simulink model "motion_controller"  (R2025b)
settings: configuration reference "MCConfiguration" (kept outside this file)
undefined symbols (not defined in the file): EstimationVelocityModes, Ts_ControlOuter, Ts_MotionController
settings Model: DataDictionary=embeddedBoard_common.sldd  VariantConfigurationObject=MCVariants  SimulationMode=accelerator  Creator=mfussi  LastModifiedBy=rpumpo
settings ConfigSetRef: SourceName=MCConfiguration

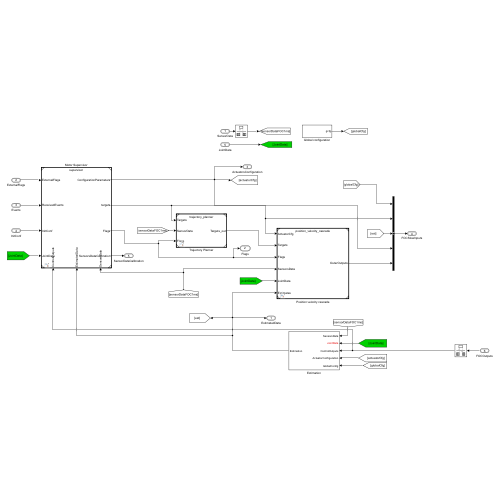
[thumbnail: Simulink's stored preview of the top-level diagram]
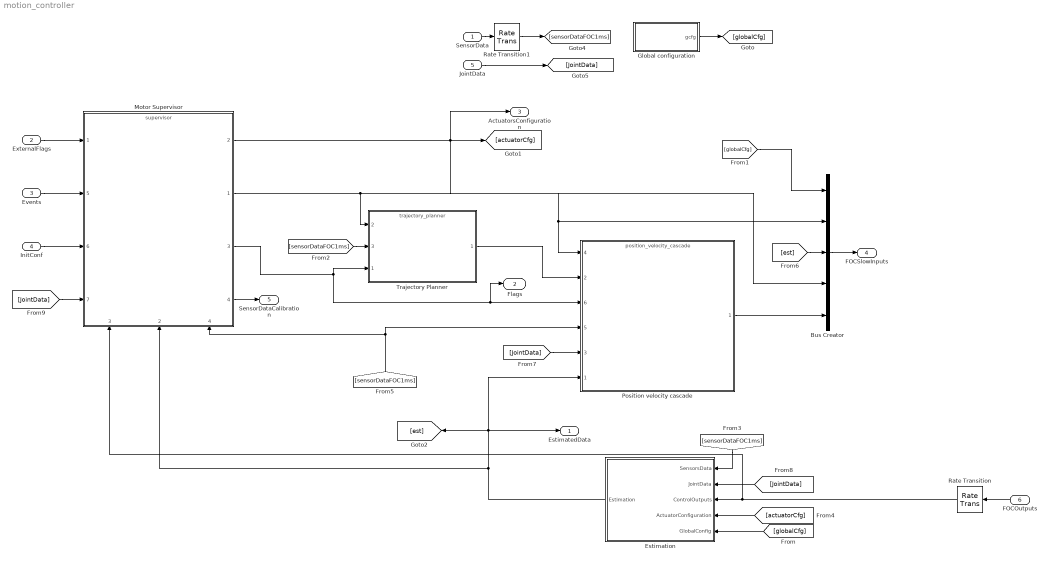
== system motion_controller ==
  SensorData : Inport  OutDataTypeStr=Bus: SensorsData  BusOutputAsStruct=on
  ExternalFlags : Inport  Port=2  OutDataTypeStr=Bus: ExternalFlags  BusOutputAsStruct=on
  Events : Inport  Port=3  OutDataTypeStr=Bus: ReceivedEvents  PortDimensions=MAX_EVENTS_PER_TICK  BusOutputAsStruct=on
  InitConf : Inport  Port=4  OutDataTypeStr=Bus: ActuatorConfiguration  BusOutputAsStruct=on
  JointData : Inport  Port=5  OutDataTypeStr=Bus: JointData  SampleTime=Ts_ControlOuter  BusOutputAsStruct=on
  FOCOutputs : Inport  Port=6  OutDataTypeStr=Bus: FOCOutputs  BusOutputAsStruct=on
  Bus Creator : BusCreator  Inputs=5  OutDataTypeStr=Bus: FOCSlowInputs  NonVirtualBus=on
      settings: InheritFromInputs=off
  Estimation : Subsystem
  Global configuration : Subsystem
  Motor Supervisor : ModelReference  ModelNameDialog=supervisor.slx  SimulationMode=Normal  ModelReferenceVersion=5.31
      settings: PortSchema="{\"entries\":[{\"content\":{\"sides\":[{\"content\":{\"connectorIds\":[\"In1\",\"In5\",\"In6\",\"In7\"]},\"type\":\"ConnectorPlacement.EquallySpacedRectSide\",\"uuid\":\"cef8e8ad-9c58-41ab-a08a-9ae722e40085\"},{\"content\":{\"connectorIds\":[\"Out2\",\"Out1\",\"Out3\",\"Out4\"],\"side\":\"RIGHT\"},\"type\":\"ConnectorPlacement.EquallySpacedRectSide\",\"uuid\":\"f0f6bf4d-d146-4c52-85d0-e4a1fe2e14c9\"},{\"content\":{\"side\":\"TOP\"},\"type\":\"ConnectorPlacement.EquallySpacedRectSide\",\"uuid\":\"118dcde8-f32d-4dec-aaf2-5a7aa823a04d\"},{\"content\":{\"connectorIds\":[\"In3\",\"In2\",\"In4\"],\"side\":\"BOTTOM\"},\"type\":\"ConnectorPlacement.EquallySpacedRectSide\",\"uuid\":\"c7cf3ffe-4331-4ad3-8d42-678750b74e71\"}]},\"type\":\"ConnectorPlacement.EquallySpacedConnector\",\"uuid\":\"5370414b-b8cf-4747-9f7c-0256206e2ab5\"}],\"packageUris\":[\"http://schema.mathworks.com/mf0/Connector/R2020b\"],\"version\":\"1.0\"}"
  Position velocity cascade : ModelReference  ModelNameDialog=position_velocity_cascade.slx  SimulationMode=Normal  ModelReferenceVersion=10.15
      settings: PortSchema="{\"entries\":[{\"content\":{\"sides\":[{\"content\":{\"connectorIds\":[\"In4\",\"In2\",\"In6\",\"In5\",\"In3\",\"In1\"]},\"type\":\"ConnectorPlacement.EquallySpacedRectSide\",\"uuid\":\"5f0855f7-78ef-4761-b7b2-78e76d92fc4b\"},{\"content\":{\"connectorIds\":[\"Out1\"],\"side\":\"RIGHT\"},\"type\":\"ConnectorPlacement.EquallySpacedRectSide\",\"uuid\":\"ce4374cd-607c-4e0b-a8af-eb2e0e17051d\"},{\"content\":{\"side\":\"TOP\"},\"type\":\"ConnectorPlacement.EquallySpacedRectSide\",\"uuid\":\"cef85d5e-e838-4f2a-8e72-80e83911c8d3\"},{\"content\":{\"side\":\"BOTTOM\"},\"type\":\"ConnectorPlacement.EquallySpacedRectSide\",\"uuid\":\"20390ec2-cce8-49cd-a78c-2a21c95dd133\"}]},\"type\":\"ConnectorPlacement.EquallySpacedConnector\",\"uuid\":\"234d6756-2ddf-48d1-9c55-249229e32550\"}],\"packageUris\":[\"http://schema.mathworks.com/mf0/Connector/R2020b\"],\"version\":\"1.0\"}"
  Rate Transition : RateTransition  Deterministic=off  OutPortSampleTime=Ts_Supervision
  Rate Transition1 : RateTransition  Deterministic=off  OutPortSampleTime=Ts_Supervision
  Trajectory Planner : ModelReference  ModelNameDialog=trajectory_planner.slx  SimulationMode=Normal  ModelReferenceVersion=2.33
      settings: PortSchema="{\"entries\":[{\"content\":{\"sides\":[{\"content\":{\"connectorIds\":[\"In2\",\"In3\",\"In1\"]},\"type\":\"ConnectorPlacement.EquallySpacedRectSide\",\"uuid\":\"9df5b159-43e0-4cee-9566-6165d3b4308e\"},{\"content\":{\"connectorIds\":[\"Out1\"],\"side\":\"RIGHT\"},\"type\":\"ConnectorPlacement.EquallySpacedRectSide\",\"uuid\":\"a479e708-d845-4af6-a357-888a4bbec164\"},{\"content\":{\"side\":\"TOP\"},\"type\":\"ConnectorPlacement.EquallySpacedRectSide\",\"uuid\":\"08bafdfa-e50b-4564-8577-557c5ee22102\"}]},\"type\":\"ConnectorPlacement.EquallySpacedConnector\",\"uuid\":\"f51dce5d-e2ef-40ca-b0ed-04a94a0f54f0\"}],\"packageUris\":[\"http://schema.mathworks.com/mf0/Connector/R2020b\"],\"version\":\"1.0\"}"
  EstimatedData : Outport  OutDataTypeStr=Bus: EstimatedData  BusOutputAsStruct=on
  Flags : Outport  Port=2  OutDataTypeStr=Bus: Flags  BusOutputAsStruct=on
  ActuatorsConfiguration : Outport  Port=3  OutDataTypeStr=Bus: ActuatorConfiguration  BusOutputAsStruct=on
  FOCSlowInputs : Outport  Port=4  OutDataTypeStr=Bus: FOCSlowInputs  BusOutputAsStruct=on
  SensorDataCalibration : Outport  Port=5  OutDataTypeStr=Bus: SensorsData  BusOutputAsStruct=on
  wires:
  Bus Creator/1 -> FOCSlowInputs/1
  Events/1 -> Motor Supervisor/5
  Motor Supervisor/1 -> Trajectory Planner/2, Bus Creator/4
  [actuatorCfg] -> Estimation/4(ActuatorConfiguration)
  FOCOutputs/1 -> Rate Transition/1
  Global configuration/1(gcfg) -> [globalCfg]
  Position velocity cascade/1 -> Bus Creator/5
  [globalCfg] -> Estimation/5(GlobalConfig)
  [globalCfg] -> Bus Creator/1
  InitConf/1 -> Motor Supervisor/6
  Motor Supervisor/2 -> ActuatorsConfiguration/1, [actuatorCfg], Position velocity cascade/4, Bus Creator/2
  ExternalFlags/1 -> Motor Supervisor/1
  [est] -> Bus Creator/3
  Motor Supervisor/3 -> Flags/1, Position velocity cascade/6, Trajectory Planner/1
  Estimation/1(Estimation) -> EstimatedData/1, Position velocity cascade/1, [est], Motor Supervisor/2
  SensorData/1 -> Rate Transition1/1
  [sensorDataFOC1ms] -> Position velocity cascade/5, Motor Supervisor/4
  [sensorDataFOC1ms] -> Estimation/1(SensorsData)
  JointData/1 -> [JointData]
  [JointData] -> Position velocity cascade/3
  [JointData] -> Estimation/2(JointData)
  [JointData] -> Motor Supervisor/7
  Rate Transition1/1 -> [sensorDataFOC1ms]
  Rate Transition/1 -> Motor Supervisor/3, Estimation/3(ControlOutputs)
  Motor Supervisor/4 -> SensorDataCalibration/1
  [sensorDataFOC1ms] -> Trajectory Planner/3
  Trajectory Planner/1 -> Position velocity cascade/2

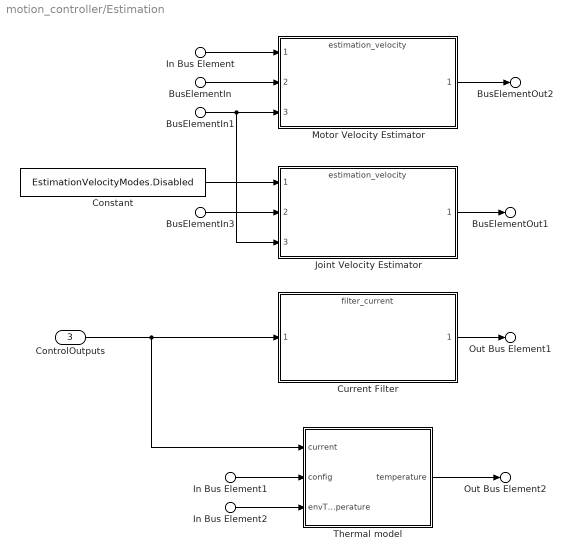
== system motion_controller/Estimation ==
  BusElementIn : Inport  Description=Mechanical Angle before gearbox  PortName=SensorsData  Element=motorsensors.qencoder.rotor_angle
  BusElementIn3 : Inport  Description=position encoder after gearbox  Port=2  PortName=JointData  Element=position
  ControlOutputs : Inport  Port=3  OutDataTypeStr=Bus: FOCOutputs
  In Bus Element1 : Inport  Port=4  PortName=ActuatorConfiguration  Element=motor
  In Bus Element2 : Inport  Port=5  PortName=GlobalConfig  Element=estimation.environment_temperature
  In Bus Element : Inport  Port=5  PortName=GlobalConfig  Element=estimation.velocity_est_mode
  BusElementIn1 : Inport  Port=5  PortName=GlobalConfig  Element=estimation.velocity_est_window
  Constant : Constant  Value=EstimationVelocityModes.Disabled  OutDataTypeStr=Enum: EstimationVelocityModes
  Current Filter : ModelReference  ModelNameDialog=filter_current.slx  SimulationMode=Normal  ModelReferenceVersion=8.0
  Joint Velocity Estimator : ModelReference  ModelNameDialog=estimation_velocity.slx  SimulationMode=Normal  ModelReferenceVersion=8.11
  Motor Velocity Estimator : ModelReference  ModelNameDialog=estimation_velocity.slx  SimulationMode=Normal  ModelReferenceVersion=8.11
  Thermal model : Subsystem  Variant=on
  BusElementOut2 : Outport  Description=velocity  PortName=Estimation  Element=rotor_velocity
  Out Bus Element1 : Outport  Description=filtered motor current  PortName=Estimation  Element=Iq_filtered
  Out Bus Element2 : Outport  Description=motor temperature  PortName=Estimation  Element=motor_temperature
  BusElementOut1 : Outport  Description=velocity  PortName=Estimation  Element=joint_velocity
  wires:
  Motor Velocity Estimator/1 -> BusElementOut2/1
  Current Filter/1 -> Out Bus Element1/1
  ControlOutputs/1 -> Current Filter/1, Thermal model/1(current)
  In Bus Element/1 -> Motor Velocity Estimator/1
  In Bus Element1/1 -> Thermal model/2(config)
  In Bus Element2/1 -> Thermal model/3(envTemperature)
  Thermal model/1(temperature) -> Out Bus Element2/1
  BusElementIn/1 -> Motor Velocity Estimator/2
  BusElementIn1/1 -> Joint Velocity Estimator/3, Motor Velocity Estimator/3
  BusElementIn3/1 -> Joint Velocity Estimator/2
  Joint Velocity Estimator/1 -> BusElementOut1/1
  Constant/1 -> Joint Velocity Estimator/1

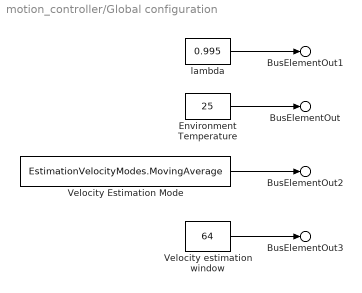
== system motion_controller/Global configuration ==
  Environment Temperature : Constant  Value=25  OutDataTypeStr=single  SampleTime=Ts_MotionController
  Velocity Estimation Mode : Constant  Value=EstimationVelocityModes.MovingAverage  OutDataTypeStr=Enum: EstimationVelocityModes  SampleTime=Ts_MotionController
  Velocity estimation window : Constant  Value=64  OutMin=1  OutDataTypeStr=uint32  SampleTime=Ts_MotionController
  lambda : Constant  Value=0.995  OutDataTypeStr=single  SampleTime=Ts_MotionController
  BusElementOut : Outport  PortName=gcfg  Element=estimation.environment_temperature
  BusElementOut1 : Outport  PortName=gcfg  Element=estimation.current_rms_lambda
  BusElementOut2 : Outport  PortName=gcfg  Element=estimation.velocity_est_mode
  BusElementOut3 : Outport  PortName=gcfg  Element=estimation.velocity_est_window
  wires:
  lambda/1 -> BusElementOut1/1
  Velocity Estimation Mode/1 -> BusElementOut2/1
  Velocity estimation window/1 -> BusElementOut3/1
  Environment Temperature/1 -> BusElementOut/1

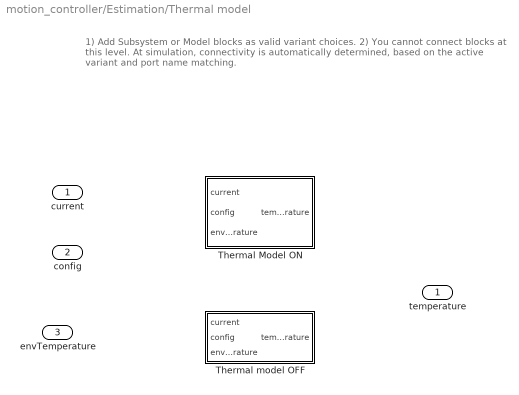
== system motion_controller/Estimation/Thermal model ==
  note: 1) Add Subsystem or Model blocks as valid variant choices.
      | 2) You cannot connect blocks at this level. At simulation, connectivity is automatically
      | determined, based on the active variant and port name matching.
  current : Inport
  config : Inport  Port=2
  envTemperature : Inport  Port=3
  Thermal Model ON : Subsystem  VariantControl=Temperature_estimation_switch == true
  Thermal model OFF : Subsystem  VariantControl=Temperature_estimation_switch == false
  temperature : Outport

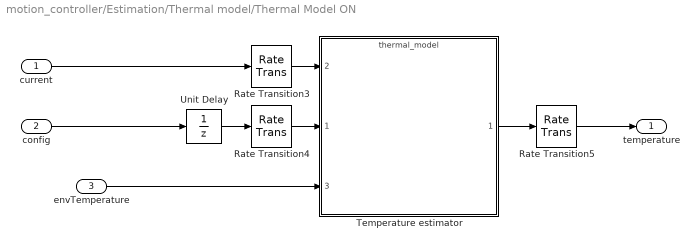
== system motion_controller/Estimation/Thermal model/Thermal Model ON ==
  current : Inport
  config : Inport  Port=2
  envTemperature : Inport  Port=3
  Rate Transition3 : RateTransition  Deterministic=off
  Rate Transition4 : RateTransition  Deterministic=off  OutPortSampleTime=1e-3
  Rate Transition5 : RateTransition  Deterministic=off
  Temperature estimator : ModelReference  ModelNameDialog=thermal_model.slx  SimulationMode=Normal  ModelReferenceVersion=8.0
      settings: PortSchema="{\"entries\":[{\"content\":{\"sides\":[{\"content\":{\"connectorIds\":[\"In2\",\"In1\",\"In3\"]},\"type\":\"ConnectorPlacement.EquallySpacedRectSide\",\"uuid\":\"78c786f4-5c3b-40e7-ad28-c0b961f14ec4\"},{\"content\":{\"connectorIds\":[\"Out1\"],\"side\":\"RIGHT\"},\"type\":\"ConnectorPlacement.EquallySpacedRectSide\",\"uuid\":\"b3487c62-68f2-43b6-a257-d51b1fb2e448\"},{\"content\":{\"side\":\"TOP\"},\"type\":\"ConnectorPlacement.EquallySpacedRectSide\",\"uuid\":\"5ce4df9e-b156-438c-989b-62dab6cef7f1\"}]},\"type\":\"ConnectorPlacement.EquallySpacedConnector\",\"uuid\":\"8f8c8caf-b0d2-4a2e-a596-6a6abf765763\"}],\"packageUris\":[\"http://schema.mathworks.com/mf0/Connector/R2020b\"],\"version\":\"1.0\"}"
  Unit Delay : UnitDelay  SampleTime=-1  HasFrameUpgradeWarning=on
  temperature : Outport
  wires:
  Rate Transition4/1 -> Temperature estimator/1
  config/1 -> Unit Delay/1
  Unit Delay/1 -> Rate Transition4/1
  Temperature estimator/1 -> Rate Transition5/1
  current/1 -> Rate Transition3/1
  Rate Transition3/1 -> Temperature estimator/2
  Rate Transition5/1 -> temperature/1
  envTemperature/1 -> Temperature estimator/3

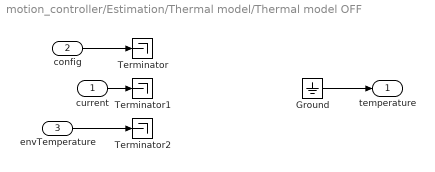
== system motion_controller/Estimation/Thermal model/Thermal model OFF ==
  current : Inport
  config : Inport  Port=2
  envTemperature : Inport  Port=3
  Ground : Ground
  Terminator : Terminator
  Terminator1 : Terminator
  Terminator2 : Terminator
  temperature : Outport
  wires:
  config/1 -> Terminator/1
  current/1 -> Terminator1/1
  envTemperature/1 -> Terminator2/1
  Ground/1 -> temperature/1
